simulink model "PFC_Full_Bridge_Unipolar_SPWM_PR"  (R2023a)
settings: Solver=FixedStepAuto  StartTime=0.0  StopTime=1  FixedStep=1e-6  RelTol=1e-3
libraries: spsMosfetLib x4, spsSeriesRLCBranchLib x3, spsVoltageMeasurementLib x2, spsACVoltageSourceLib x1, spsCurrentMeasurementLib x1, spsMeanLib x1, slpidlib x1, powerlib_extras x1, spsTHDLib x1, spspowerguiLib x1, simulink x1
settings Model: SimulationMode=accelerator  Creator=ZhuanZ（无密码）  LastModifiedBy=Qu

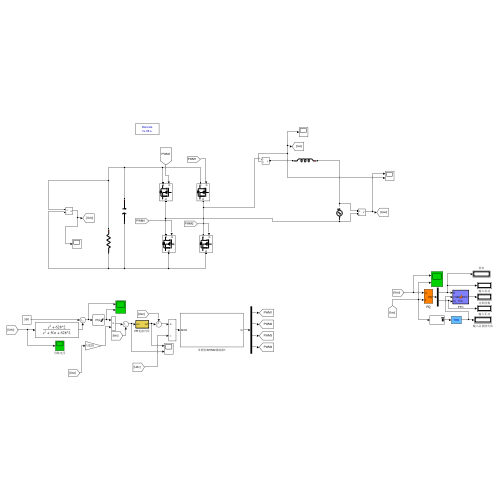
[thumbnail: Simulink's stored preview of the top-level diagram]
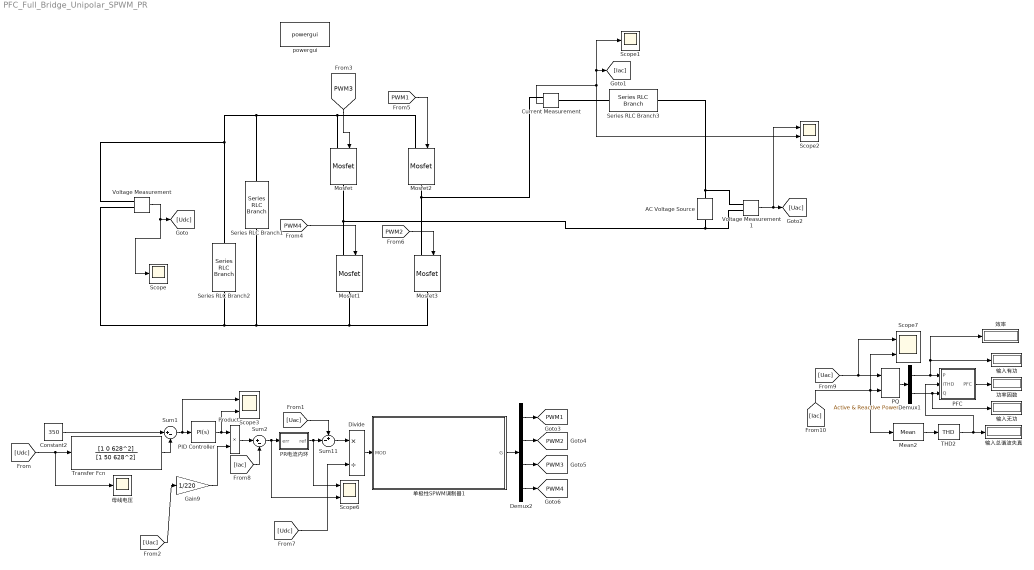
== system PFC_Full_Bridge_Unipolar_SPWM_PR ==
  AC Voltage Source : spsACVoltageSourceLib/AC Voltage Source  Amplitude=311  Phase=0  Frequency=50  SampleTime=0  Measurements=None  BusType=swing  Pref=10e3  Qref=0  Qmin=-inf  Qmax=+inf
  Constant2 : Constant  Value=350
  Current Measurement : spsCurrentMeasurementLib/Current Measurement  PhasorSimulation=off  OutputType=Complex  PSBequivalent=0
  Demux1 : Demux  Outputs=2
  Demux2 : Demux
  Divide : Product  Inputs=*/
  Gain9 : Gain  Gain=1/220
  Mean2 : spsMeanLib/Mean  Freq=10000  Vinit=0  Ts=0
  Mosfet : spsMosfetLib/Mosfet  Ron=0.05  Lon=0  Rd=0.01  Vfd=1  IC=0  Rs=1e5  Cs=inf  Measurements=off
  Mosfet1 : spsMosfetLib/Mosfet  Ron=0.05  Lon=0  Rd=0.01  Vfd=1  IC=0  Rs=1e5  Cs=inf  Measurements=off
  Mosfet2 : spsMosfetLib/Mosfet  Ron=0.05  Lon=0  Rd=0.01  Vfd=1  IC=0  Rs=1e5  Cs=inf  Measurements=off
  Mosfet3 : spsMosfetLib/Mosfet  Ron=0.050  Lon=0  Rd=0.01  Vfd=1  IC=0  Rs=1e5  Cs=inf  Measurements=off
  PFC : MATLAB Function  TreatAsAtomicUnit=on
  PID Controller : slpidlib/PID Controller  Controller=PI  Form=Parallel  TimeDomain=Continuous-time  UseExternalTs=off  SampleTime=-1  IntegratorMethod=Forward Euler  FilterMethod=Forward Euler  ControllerParametersSource=internal  P=0.4  I=10  UseKiTs=off  D=0.001  N=100  UseFilter=on  TunerSelectOption=Transfer Function Based (PID Tuner App)  InitialConditionSource=internal  InitialConditionForIntegrator=0  InitialConditionForFilter=0  DifferentiatorICPrevScaledInput=0  ExternalReset=none  TrackingMode=off  Kt=1  LimitOutput=on  SatLimitsSource=internal  UpperSaturationLimit=200  LowerSaturationLimit=-200  LinearizeAsGain=on  AntiWindupMode=clamping  Kb=1  LimitIntegrator=off  UpperIntegratorSaturationLimit=inf  LowerIntegratorSaturationLimit=-inf  POutMin=[]  POutMax=[]  IOutMin=[]  IOutMax=[]  DOutMin=[]  DOutMax=[]  NOutMin=[]  NOutMax=[]  SumOutMin=[]  SumOutMax=[]  SaturationOutMin=[]  SaturationOutMax=[]  PParamMin=[]  PParamMax=[]  IParamMin=[]  IParamMax=[]  DParamMin=[]  DParamMax=[]  NParamMin=[]  NParamMax=[]  KbParamMin=[]  KbParamMax=[]  KtParamMin=[]  KtParamMax=[]  KbOutMin=[]  KbOutMax=[]  KtOutMin=[]  KtOutMax=[]  IntegratorOutMin=[]  IntegratorOutMax=[]  FilterOutMin=[]  FilterOutMax=[]  SumI1OutMin=[]  SumI1OutMax=[]  SumI2OutMin=[]  SumI2OutMax=[]  SumI3OutMin=[]  SumI3OutMax=[]  SumI4OutMin=[]  SumI4OutMax=[]  SumDOutMin=[]  SumDOutMax=[]  DifferentiatorOutMin=[]  DifferentiatorOutMax=[]  FilterDiffOutCoefMin=[]  FilterDiffOutCoefMax=[]  ReciprocalOutMin=[]  ReciprocalOutMax=[]  SumDenOutMin=[]  SumDenOutMax=[]  SumNumOutMin=[]  SumNumOutMax=[]  DivideOutMin=[]  DivideOutMax=[]  UdiffTsProdOutMin=[]  UdiffTsProdOutMax=[]  NTsProdOutMin=[]  NTsProdOutMax=[]  UintegralTsProdOutMin=[]  UintegralTsProdOutMax=[]  UngainTsProdOutMin=[]  UngainTsProdOutMax=[]  ClampingZeroOutDataTypeStr=Inherit: Inherit via back propagation  ClampingZeroOutMin=[]  ClampingZeroOutMax=[]  FilterDenConstantOutDataTypeStr=Inherit: Inherit via back propagation  FilterDenConstantOutMin=[]  FilterDenConstantOutMax=[]  PCopyOutDataTypeStr=Inherit: Inherit via back propagation  PCopyOutMin=[]  PCopyOutMax=[]  NCopyOutDataTypeStr=Inherit: Inherit via back propagation  NCopyOutMin=[]  NCopyOutMax=[]  IntegratorContinuousStateAttributes=''  IntegratorStateMustResolveToSignalObject=off  IntegratorRTWStateStorageClass=Auto  FilterContinuousStateAttributes=''  FilterStateMustResolveToSignalObject=off  FilterRTWStateStorageClass=Auto  ParallelPVariant=InternalParameters  IdealPVariant=Disabled  IVariant=InternalParameters  DVariant=Disabled  IntegratorVariant=Continuous  SatVariant=Enabled  AWVariant=ContClampingParallel  PCopyVariant=Disabled  TRVariant=Disabled  FdbkBlocksVariant=Forward  IdealPFdbkVariant=Disabled  SatFdbkVariant=Disabled  DerivativeFilterVariant=Disabled  NVariant=Disabled  NCopyVariant=Disabled_SignalSpec  FilterICVariant=Disabled  IntegratorICVariant=InternalICs  ExternalResetVariant=Disabled  TRSumVariant=Passthrough  SumFdbkVariant=Disabled  SumVariant=Sum_PI  TsampFilterVariant=InternalTs  TsampNgainVariant=Passthrough  TsampIntegralVariant=Disabled_SignalSpec  ExternalSaturationOutDataTypeStr=Inherit: Same as second input
  PQ : powerlib_extras/Measurements/Active & Reactive Power  f1=50
  PR电流内环 : Subsystem  TreatAsAtomicUnit=on  mask{Kp=3, Kr=100, Wc=5, Upper=310, Lower=-310}
  Product : Product
  Scope : Scope
  Scope1 : Scope
  Scope{2..3,6..7} (4 alike) : Scope  NumInputPorts=2
  Series RLC Branch1 : spsSeriesRLCBranchLib/Series RLC Branch  LConnTagsString=__new0  RConnTagsString=__new0  BranchType=C  Resistance=1  Inductance=1e-3  SetiL0=off  InitialCurrent=0  Capacitance=4e-3  Setx0=on  InitialVoltage=310  Measurements=None
  Series RLC Branch2 : spsSeriesRLCBranchLib/Series RLC Branch  LConnTagsString=__new0  RConnTagsString=__new0  BranchType=R  Resistance=25  Inductance=1e-3  SetiL0=off  InitialCurrent=0  Capacitance=4e-3  Setx0=on  InitialVoltage=310  Measurements=None
  Series RLC Branch3 : spsSeriesRLCBranchLib/Series RLC Branch  LConnTagsString=__new0  RConnTagsString=__new0  BranchType=L  Resistance=50  Inductance=6e-4  SetiL0=off  InitialCurrent=0  Capacitance=1e-6  Setx0=off  InitialVoltage=0  Measurements=None
  Sum1 : Sum  Inputs=|+-
  Sum11 : Sum  Inputs=+-|
  Sum2 : Sum  Inputs=|+-
  THD2 : spsTHDLib/THD  Freq=50  Ts=0
  Transfer Fcn : TransferFcn  Numerator=[1 0 628^2]  Denominator=[1 50 628^2]
  Voltage Measurement : spsVoltageMeasurementLib/Voltage Measurement  PhasorSimulation=off  OutputType=Complex  PSBequivalent=0
  Voltage Measurement1 : spsVoltageMeasurementLib/Voltage Measurement  PhasorSimulation=off  OutputType=Complex  PSBequivalent=0
  powergui : spspowerguiLib/powergui  Priority=1  SimulationMode=Discrete  SampleTime=1e-6  frequency=60  Iterations=50  frequencyindice=50  Pbase=100e6  ErrMax=1e-4  UnitsV=kV  UnitsW=MW  buscounter=0  FunctionMessages=off  echomessages=off  EnableUseOfTLC=off  CurrentSourceSwitches=off  DisableSnubberDevices=off  DisableRonSwitches=off  DisableVfSwitches=off  DisplayEquations=off  AutomaticDiscreteSolvers=off  SolverType=Tustin/Backward Euler (TBE)  Interpol=off  ExternalGateDelay=off  methode=off  Ts=100  x0status=blocks  SPID=on  SwTol=0  HookPort=off  NonlinearTolerance=1e-4  nMaxIteration=100  ContinueOnMaxIteration=off  RestoreLinks=warning  ResistiveCurrentMeasurement=off  Frange=[0:2:500]  Ylog=off  Xlog=on  ShowGrid=off  save=off  variable=ZData  structure=0  ZoomFFT=off  StartTime=0.0  cycles=1  DisplayStyle=1  fundamental=60  FreqAxis=off  MaxFrequency=1000  frequencyindicesteady=1  RmsSteady=1  display=off
  功率因数 : Display
  单极性SPWM调制器1 : Subsystem
  效率 : Display
  母线电压 : Scope
  输入总谐波失真 : Display
  输入无功 : Display
  输入有功 : Display
  tag scope: PWM1=global, PWM2=global, PWM3=global, PWM4=global
  wires:
  Voltage Measurement/1 -> Scope/1, [Udc]
  Current Measurement/1 -> Scope2/2, Scope1/1, [Iac]
  Voltage Measurement1/1 -> Scope2/1, [Uac]
  [PWM3] -> Mosfet/1
  [PWM4] -> Mosfet1/1
  [PWM1] -> Mosfet2/1
  [PWM2] -> Mosfet3/1
  Demux1/1 -> 效率/1, 输入有功/1, PFC/1(P)
  [Iac] -> Mean2/1, PQ/2, Scope7/2
  [Uac] -> PQ/1, Scope7/1
  PQ/1 -> Demux1/1
  THD2/1 -> 输入总谐波失真/1, PFC/2(iTHD)
  PFC/1(PFC) -> 功率因数/1
  Mean2/1 -> THD2/1
  Demux1/2 -> 输入无功/1, PFC/3(Q)
  PR电流内环/1(ref) -> Scope6/1, Sum11/2
  Sum1/1 -> Scope3/1, PID Controller/1
  [Iac] -> Sum2/2
  Product/1 -> Sum2/1
  Gain9/1 -> Product/2
  Sum2/1 -> Scope6/2, PR电流内环/1(err)
  Transfer Fcn/1 -> Sum1/2
  Demux2/3 -> [PWM3]
  Constant2/1 -> Sum1/1
  [Uac] -> Gain9/1
  [Uac] -> Sum11/1
  Divide/1 -> 单极性SPWM调制器1/1(MOD)
  Demux2/2 -> [PWM2]
  [Udc] -> Divide/2
  Sum11/1 -> Divide/1
  PID Controller/1 -> Scope3/2, Product/1
  Demux2/4 -> [PWM4]
  单极性SPWM调制器1/1(G) -> Demux2/1
  [Udc] -> Transfer Fcn/1, 母线电压/1
  Demux2/1 -> [PWM1]
  connections:
  Mosfet/LConn1 -- Series RLC Branch2/LConn1 -- Voltage Measurement/LConn1 -- Series RLC Branch1/LConn1 -- Mosfet2/LConn1
  Mosfet1/RConn1 -- Series RLC Branch2/RConn1 -- Voltage Measurement/LConn2 -- Series RLC Branch1/RConn1 -- Mosfet3/RConn1
  Voltage Measurement1/LConn2 -- Mosfet1/LConn1 -- Mosfet/RConn1 -- AC Voltage Source/LConn1
  Mosfet2/RConn1 -- Current Measurement/RConn1 -- Mosfet3/LConn1
  Series RLC Branch3/LConn1 -- Voltage Measurement1/LConn1 -- AC Voltage Source/RConn1
  Series RLC Branch3/RConn1 -- Current Measurement/LConn1

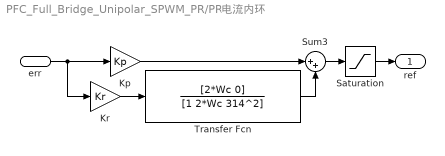
== system PFC_Full_Bridge_Unipolar_SPWM_PR/PR电流内环 ==
  err : Inport
  Kp : Gain  Gain=Kp
  Kr : Gain  Gain=Kr
  Saturation : Saturate  UpperLimit=Upper  LowerLimit=Lower
  Sum3 : Sum  Inputs=|++
  Transfer Fcn : TransferFcn  Numerator=[2*Wc 0]  Denominator=[1 2*Wc 314^2]
  ref : Outport
  wires:
  Kp/1 -> Sum3/1
  Kr/1 -> Transfer Fcn/1
  Transfer Fcn/1 -> Sum3/2
  Saturation/1 -> ref/1
  err/1 -> Kr/1, Kp/1
  Sum3/1 -> Saturation/1

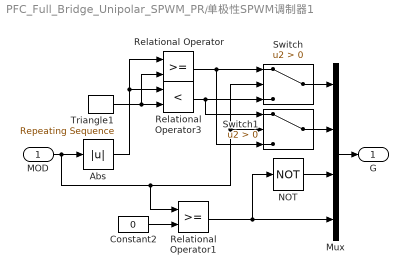
== system PFC_Full_Bridge_Unipolar_SPWM_PR/单极性SPWM调制器1 ==
  MOD : Inport
  Abs : Abs  SaturateOnIntegerOverflow=off
  Constant2 : Constant  Value=0
  Mux : Mux
  NOT : Logic  Operator=NOT  IconShape=distinctive  AllPortsSameDT=off  OutDataTypeStr=boolean
  Relational Operator : RelationalOperator  OutDataTypeStr=boolean  InputSameDT=off
  Relational Operator1 : RelationalOperator  OutDataTypeStr=boolean  InputSameDT=off
  Relational Operator3 : RelationalOperator  Operator=<  OutDataTypeStr=boolean  InputSameDT=off
  Switch : Switch  Criteria=u2 > Threshold  SaturateOnIntegerOverflow=off  InputSameDT=off
  Switch1 : Switch  Criteria=u2 > Threshold  SaturateOnIntegerOverflow=off  InputSameDT=off
  Triangle1 : simulink/Sources/Repeating Sequence  rep_seq_t=[0 1/20000/2 1/20000]  rep_seq_y=[0 1 0]
  G : Outport
  wires:
  NOT/1 -> Mux/3
  Constant2/1 -> Relational Operator1/2
  Relational Operator1/1 -> NOT/1, Mux/4
  Abs/1 -> Relational Operator3/1, Relational Operator/1
  MOD/1 -> Abs/1, Relational Operator1/1, Switch/2, Switch1/2
  Mux/1 -> G/1
  Triangle1/1 -> Relational Operator3/2, Relational Operator/2
  Relational Operator/1 -> Switch1/3, Switch/1
  Switch/1 -> Mux/1
  Switch1/1 -> Mux/2
  Relational Operator3/1 -> Switch/3, Switch1/1

== matlab function PFC_Full_Bridge_Unipolar_SPWM_PR/PFC ==
  data: P input; iTHD input; PFC output; Q input
function PFC = fcn(P,iTHD,Q)
% This block supports an embeddable subset of the MATLAB language.
% See the help menu for details. 
PFC=(P/sqrt(P*P+Q*Q))/sqrt(1+iTHD*iTHD);
